simulink model "uacs_flight_bench_en"  (R2024a)
settings: Solver=ode4  StartTime=0.0  StopTime=sim_bench_t_end  FixedStep=sim_ts_ctrl  RelTol=1e-3
PreLoadFcn:
  | p=fileparts(fileparts(get_param(bdroot,'FileName')));addpath(p,fullfile(p,'params'),fullfile(p,'plant'),fullfile(p,'control'),fullfile(p,'sim'),fullfile(p,'run'),fullfile(p,'verify'),'-begin');uacs_go
PostLoadFcn:
  | uacs_bench_seed_en('uacs_flight_bench_en')
InitFcn:
  | p=fileparts(fileparts(get_param(bdroot,'FileName')));addpath(p,fullfile(p,'params'),fullfile(p,'plant'),fullfile(p,'control'),fullfile(p,'sim'),fullfile(p,'run'),fullfile(p,'verify'),'-begin');uacs_ensure
StopFcn:
  | uacs_bench_record('uacs_flight_bench_en')
undefined symbols (not defined in the file): DiscIntNeverNeededParam, sim_alpha_stall_abs, sim_c_neg1, sim_c_zero, sim_dist_gust_amp, sim_dist_gust_dir, sim_dist_gust_freq, sim_dist_wind_ned, sim_G_surf, sim_js_pitch_sign, sim_lqr_C_lat, sim_lqr_C_long, sim_lqr_K_lat, sim_lqr_K_long, sim_lqr_Tref_lat, sim_lqr_Tref_long, sim_lqr_Uff_lat, sim_lqr_Uff_long, sim_lqr_xop_lat, sim_lqr_xop_long, sim_lqr_zlim_lat, sim_lqr_zlim_lat_neg, sim_lqr_zlim_long, sim_lqr_zlim_long_neg, sim_pid_h_Dden, sim_pid_h_Dnum_abs, sim_pid_h_Isat, sim_pid_h_Isat_neg, sim_pid_h_Kp_abs, sim_pid_h_lim, sim_pid_h_lim_neg, sim_pid_h_pol, sim_pid_h_Ts, sim_pid_p_Dden, sim_pid_p_Dnum_abs, sim_pid_p_Isat, sim_pid_p_Isat_neg, sim_pid_p_Kp_abs, sim_pid_p_pol, sim_pid_p_Ts, sim_pid_phi_Dden, sim_pid_phi_Dnum_abs, sim_pid_phi_Isat, sim_pid_phi_Isat_neg, sim_pid_phi_Kp_abs, sim_pid_phi_pol, sim_pid_phi_Ts, sim_pid_q_Dden, sim_pid_q_Dnum_abs, sim_pid_q_Isat, sim_pid_q_Isat_neg, sim_pid_q_Kp_abs, sim_pid_q_pol, sim_pid_q_Ts, sim_pid_r_Dden, sim_pid_r_Dnum_abs, sim_pid_r_Isat, sim_pid_r_Isat_neg, sim_pid_r_Kp_abs, sim_pid_r_pol ... (+22)
libraries: aerolibanimutils x1
settings Model: Creator=Ash Trailer  LastModifiedBy=Ash Trailer
settings DataIOCC: SaveFormat=StructureWithTime
settings DebuggingCC: AlgebraicLoopMsg=error

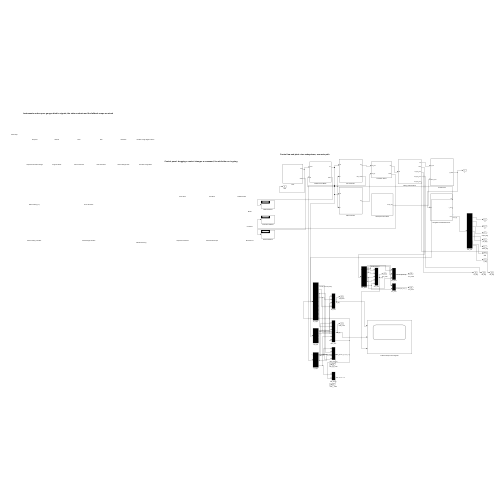
[thumbnail: Simulink's stored preview of the top-level diagram]
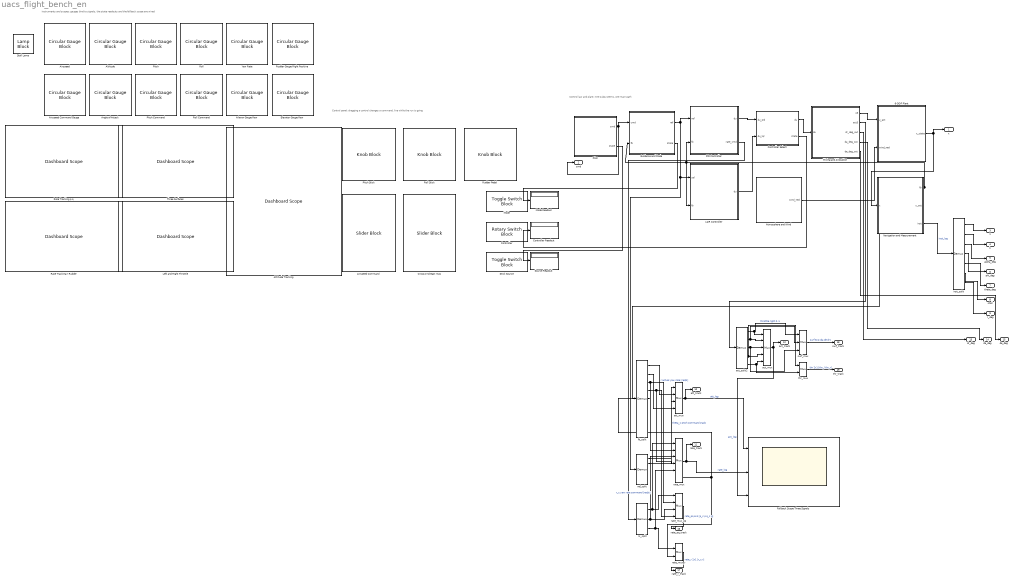
== system uacs_flight_bench_en ==
  note: Control panel: dragging a control changes a command, live while the run is going
  note: Control law and plant: nine subsystems, one main path
  note: Instruments and scopes: gauges bind to signals, the state readouts and the fallback scope are wired
  6-DOF Plant : Subsystem
  Aileron Gauge Raw : CircularGaugeBlock  ScaleMin=-30  ScaleMax=30
  Airspeed : CircularGaugeBlock  ScaleMax=40
  Airspeed Command : SliderBlock  ScaleMax=1
  Airspeed Command Gauge : CircularGaugeBlock  ScaleMax=40
  Altitude : CircularGaugeBlock  ScaleMax=400
  Angle of Attack : CircularGaugeBlock  ScaleMin=-15  ScaleMax=20
  Atmosphere and Wind : Subsystem
  Attitude Tracking : DashboardScope
  Controller : RotarySwitchBlock
      settings: Values={{'PID', 'LQR'}, [0 1]}
  Controller Readout : Display
  Controller Select : Subsystem
  Crosswind East mps : SliderBlock  ScaleMin=-10  ScaleMax=10
  Elevator Gauge Raw : CircularGaugeBlock  ScaleMin=-30  ScaleMax=30
  Fallback Scope Three Signals : Scope  NumInputPorts=3
  Guidance and Mode : Subsystem
  LQR Controller : Subsystem
  Left and Right Throttle : DashboardScope
  Mixing and Allocation : Subsystem
  Mode : ToggleSwitchBlock
      settings: Values={{'Attitude', 'Altitude'}, [0 1]}
  Mode Readout : Display
  Navigation and Measurement : Subsystem
  PID Controller : Subsystem
  Pilot : Subsystem
  Pitch : CircularGaugeBlock  ScaleMin=-30  ScaleMax=30
  Pitch Command : CircularGaugeBlock  ScaleMin=-30  ScaleMax=30
  Pitch Stick : KnobBlock  ScaleMin=-1  ScaleMax=1
  Rate Tracking p q : DashboardScope
  Rate Tracking r Rudder : DashboardScope
  Roll : CircularGaugeBlock  ScaleMin=-60  ScaleMax=60
  Roll Command : CircularGaugeBlock  ScaleMin=-60  ScaleMax=60
  Roll Stick : KnobBlock  ScaleMin=-1  ScaleMax=1
  Rudder Gauge Right Positive : CircularGaugeBlock  ScaleMin=-30  ScaleMax=30
  Rudder Pedal : KnobBlock  ScaleMin=-1  ScaleMax=1
  Source Readout : Display
  Stall Lamp : LampBlock
  Stick Source : ToggleSwitchBlock
      settings: Values={{'Virtual stick', 'Gamepad'}, [0 1]}
  Three Surfaces : DashboardScope
  Yaw Rate : CircularGaugeBlock  ScaleMin=-60  ScaleMax=60
  act_mux : Mux  Inputs=5
  act_split2 : Demux  Outputs=5
  att_mux : Mux
  fb_split : Demux  Outputs=9
  inst_split : Demux  Outputs=7
  rate_mux : Mux  Inputs=6
  rate_mux_pq : Mux
  rate_mux_r : Mux  Inputs=2
  rc_split : Demux  Outputs=3
  ref_split : Demux  Outputs=5
  surf_mux : Mux  Inputs=3
  thr_mux : Mux  Inputs=2
  x : Outport
  cmd : Outport  Port=2
  V : Outport  Port=3
  h : Outport  Port=4
  alpha_deg : Outport  Port=5
  phi_deg : Outport  Port=6
  theta_deg : Outport  Port=7
  stall : Outport  Port=8
  r_deg : Outport  Port=9
  att_track : Outport  Port=10
  rate_track : Outport  Port=11
  act_track : Outport  Port=12
  dr_deg : Outport  Port=13
  da_deg : Outport  Port=14
  de_deg : Outport  Port=15
  rate_pq_track : Outport  Port=16
  rate_r_track : Outport  Port=17
  surf_track : Outport  Port=18
  thr_track : Outport  Port=19
  wires:
  Pilot/1(cmd) -> Guidance and Mode/1(cmd), cmd/1
  Navigation and Measurement/1(fb) -> Guidance and Mode/2(fb), PID Controller/2(fb), LQR Controller/2(fb), fb_split/1
  Guidance and Mode/1(ref) -> ref_split/1, LQR Controller/1(ref), PID Controller/1(ref)
  PID Controller/1(du) -> Controller Select/1(du_pid)
  LQR Controller/1(du) -> Controller Select/2(du_lqr)
  Controller Select/1(du) -> Mixing and Allocation/1(du)
  Mixing and Allocation/1(u6) -> 6-DOF Plant/1(u_act)
  Atmosphere and Wind/1(wind_ned) -> 6-DOF Plant/2(wind_ned)
  6-DOF Plant/1(x_state) -> Navigation and Measurement/1(x), x/1
  Guidance and Mode/2(state) -> Mode Readout/1
  Controller Select/2(state) -> Controller Readout/1
  Pilot/2(state) -> Source Readout/1
  PID Controller/2(rate_cmd) -> rc_split/1
  Navigation and Measurement/3(inst) -> inst_split/1  "inst_log"
  inst_split/1 -> V/1
  inst_split/2 -> h/1
  inst_split/3 -> alpha_deg/1
  inst_split/4 -> phi_deg/1
  inst_split/5 -> theta_deg/1
  inst_split/6 -> stall/1
  inst_split/7 -> r_deg/1
  ref_split/1 -> att_mux/1  "theta_c pitch command [rad]"
  fb_split/1 -> att_mux/2  "r actual yaw rate [rad/s]"
  ref_split/2 -> att_mux/3
  fb_split/2 -> att_mux/4
  att_mux/1 -> Fallback Scope Three Signals/1, att_track/1  "att_log"
  rc_split/1 -> rate_mux/1, rate_mux_pq/1  "r_c yaw rate command [rad/s]"
  fb_split/3 -> rate_mux_pq/2, rate_mux/2
  rc_split/2 -> rate_mux/3, rate_mux_pq/3
  fb_split/4 -> rate_mux_pq/4, rate_mux/4
  rc_split/3 -> rate_mux/5, rate_mux_r/1
  fb_split/5 -> rate_mux_r/2, rate_mux/6
  rate_mux/1 -> Fallback Scope Three Signals/2, rate_track/1  "rate_log"
  Mixing and Allocation/2(act5) -> act_split2/1
  act_split2/1 -> surf_mux/1, act_mux/1  "throttle right 0..1"
  act_split2/2 -> surf_mux/2, act_mux/2
  act_split2/3 -> act_mux/3, surf_mux/3
  act_split2/4 -> act_mux/4, thr_mux/1
  act_split2/5 -> act_mux/5, thr_mux/2
  act_mux/1 -> Fallback Scope Three Signals/3, act_track/1  "act_log"
  Mixing and Allocation/3(dr_deg_out) -> dr_deg/1
  Mixing and Allocation/4(da_deg_out) -> da_deg/1
  Mixing and Allocation/5(de_deg_out) -> de_deg/1
  rate_mux_pq/1 -> rate_pq_track/1  "rate_pq 4x1 [p_c p q_c q]"
  rate_mux_r/1 -> rate_r_track/1  "rate_r 2x1 [r_c r]"
  surf_mux/1 -> surf_track/1  "surf 3x1 [da de dr]"
  thr_mux/1 -> thr_track/1  "thr 2x1 [thr_l thr_r]"

== system uacs_flight_bench_en/6-DOF Plant ==
  u_act : Inport
  wind_ned : Inport  Port=2
  plant_eom : M-S-Function  FunctionName=sim_plant_sfun
  x_state : Outport
  wires:
  u_act/1 -> plant_eom/1
  wind_ned/1 -> plant_eom/2
  plant_eom/1 -> x_state/1

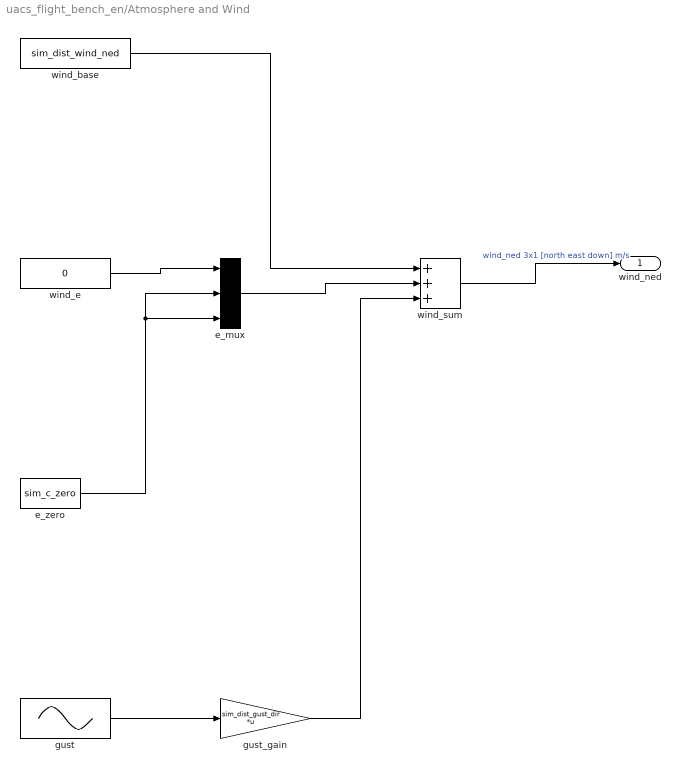
== system uacs_flight_bench_en/Atmosphere and Wind ==
  e_mux : Mux  Inputs=3
  e_zero : Constant  Value=sim_c_zero
  gust : Sin  Amplitude=sim_dist_gust_amp  Frequency=sim_dist_gust_freq  SampleTime=0
  gust_gain : Gain  Gain=sim_dist_gust_dir  Multiplication=Matrix(K*u)
  wind_base : Constant  Value=sim_dist_wind_ned
  wind_e : Constant  Value=0
  wind_sum : Sum  Inputs=+++
  wind_ned : Outport
  wires:
  wind_e/1 -> e_mux/1
  e_zero/1 -> e_mux/2, e_mux/3
  wind_base/1 -> wind_sum/1
  e_mux/1 -> wind_sum/2
  gust/1 -> gust_gain/1
  gust_gain/1 -> wind_sum/3
  wind_sum/1 -> wind_ned/1  "wind_ned 3x1 [north east down] m/s"

== system uacs_flight_bench_en/Controller Select ==
  du_pid : Inport
  du_lqr : Inport  Port=2
  k_sel : Constant  Value=0
  sw : Switch  Criteria=u2 ~= 0  Threshold=sim_c_zero  SaturateOnIntegerOverflow=off  InputSameDT=off
  du : Outport
  state : Outport  Port=2
  wires:
  du_lqr/1 -> sw/1  "1 LQR"
  k_sel/1 -> sw/2, state/1
  du_pid/1 -> sw/3  "0 PID"
  sw/1 -> du/1

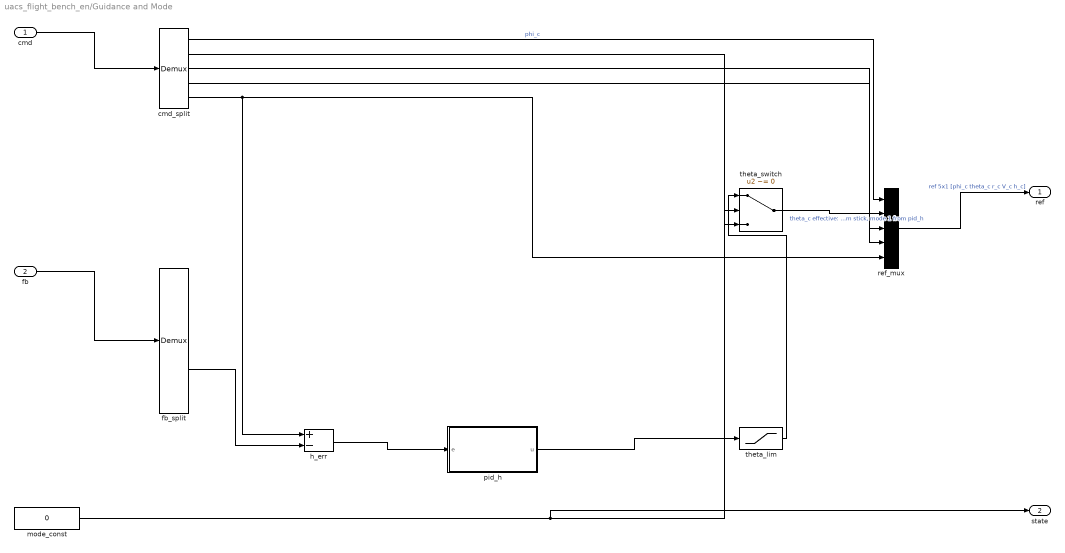
== system uacs_flight_bench_en/Guidance and Mode ==
  cmd : Inport
  fb : Inport  Port=2
  cmd_split : Demux  Outputs=5
  fb_split : Demux  Outputs=9
  h_err : Sum  Inputs=+-
  mode_const : Constant  Value=0
  pid_h : Subsystem
  ref_mux : Mux  Inputs=5
  theta_lim : Saturate  UpperLimit=sim_pid_h_lim  LowerLimit=sim_pid_h_lim_neg
  theta_switch : Switch  Criteria=u2 ~= 0  Threshold=sim_c_zero  SaturateOnIntegerOverflow=off  InputSameDT=off
  ref : Outport
  state : Outport  Port=2
  wires:
  cmd/1 -> cmd_split/1
  fb/1 -> fb_split/1
  cmd_split/5 -> h_err/1, ref_mux/5
  fb_split/7 -> h_err/2
  h_err/1 -> pid_h/1(e)
  pid_h/1(u) -> theta_lim/1
  theta_lim/1 -> theta_switch/1
  mode_const/1 -> theta_switch/2, state/1
  cmd_split/2 -> theta_switch/3
  cmd_split/1 -> ref_mux/1  "phi_c"
  theta_switch/1 -> ref_mux/2  "theta_c effective: mode 0 from stick, mode 1 from pid_h"
  cmd_split/3 -> ref_mux/3
  cmd_split/4 -> ref_mux/4
  ref_mux/1 -> ref/1  "ref 5x1 [phi_c theta_c r_c V_c h_c]"

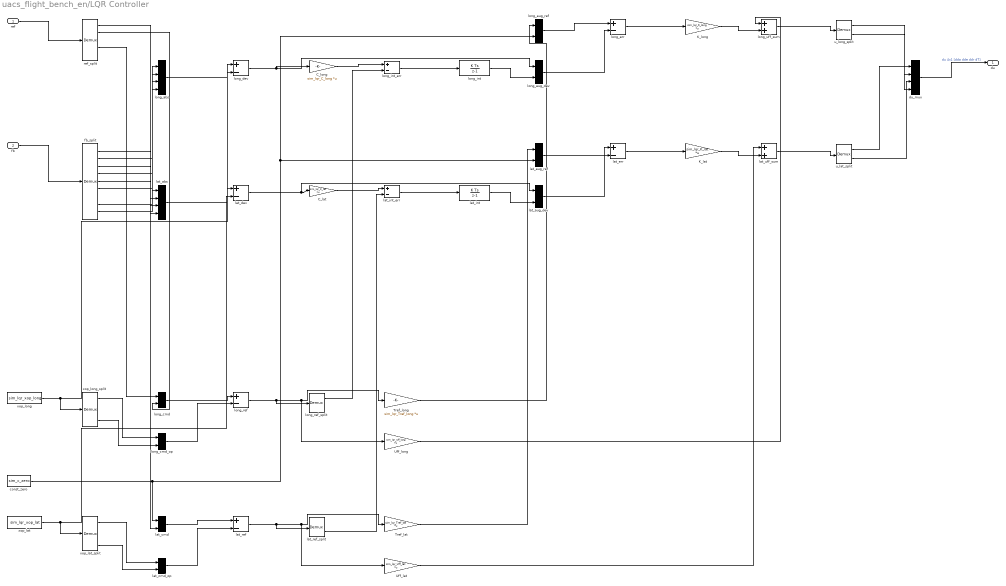
== system uacs_flight_bench_en/LQR Controller ==
  ref : Inport
  fb : Inport  Port=2
  C_lat : Gain  Gain=sim_lqr_C_lat  Multiplication=Matrix(K*u)
  C_long : Gain  Gain=sim_lqr_C_long  Multiplication=Matrix(K*u)
  K_lat : Gain  Gain=sim_lqr_K_lat  Multiplication=Matrix(K*u)
  K_long : Gain  Gain=sim_lqr_K_long  Multiplication=Matrix(K*u)
  Tref_lat : Gain  Gain=sim_lqr_Tref_lat  Multiplication=Matrix(K*u)
  Tref_long : Gain  Gain=sim_lqr_Tref_long  Multiplication=Matrix(K*u)
  Uff_lat : Gain  Gain=sim_lqr_Uff_lat  Multiplication=Matrix(K*u)
  Uff_long : Gain  Gain=sim_lqr_Uff_long  Multiplication=Matrix(K*u)
  const_zero : Constant  Value=sim_c_zero
  du_mux : Mux
  fb_split : Demux  Outputs=9
  lat_abs : Mux
  lat_aug_dev : Mux  Inputs=2
  lat_aug_ref : Mux  Inputs=2
  lat_cmd : Mux  Inputs=2
  lat_cmd_op : Mux  Inputs=2
  lat_dev : Sum  Inputs=+-
  lat_err : Sum  Inputs=+-
  lat_int : DiscreteIntegrator  gainval=sim_c_one  SampleTime=sim_ts_ctrl  LimitOutput=on  UpperSaturationLimit=sim_lqr_zlim_lat  LowerSaturationLimit=sim_lqr_zlim_lat_neg  ICPrevOutput=DiscIntNeverNeededParam  ICPrevScaledInput=DiscIntNeverNeededParam
  lat_int_err : Sum  Inputs=+-
  lat_ref : Sum  Inputs=+-
  lat_ref_split : Demux  Outputs=2
  lat_uff_sum : Sum
  long_abs : Mux
  long_aug_dev : Mux  Inputs=2
  long_aug_ref : Mux  Inputs=2
  long_cmd : Mux  Inputs=2
  long_cmd_op : Mux  Inputs=2
  long_dev : Sum  Inputs=+-
  long_err : Sum  Inputs=+-
  long_int : DiscreteIntegrator  gainval=sim_c_one  SampleTime=sim_ts_ctrl  LimitOutput=on  UpperSaturationLimit=sim_lqr_zlim_long  LowerSaturationLimit=sim_lqr_zlim_long_neg  ICPrevOutput=DiscIntNeverNeededParam  ICPrevScaledInput=DiscIntNeverNeededParam
  long_int_err : Sum  Inputs=+-
  long_ref : Sum  Inputs=+-
  long_ref_split : Demux  Outputs=2
  long_uff_sum : Sum
  ref_split : Demux  Outputs=5
  u_lat_split : Demux  Outputs=2
  u_long_split : Demux  Outputs=2
  xop_lat : Constant  Value=sim_lqr_xop_lat
  xop_lat_split : Demux
  xop_long : Constant  Value=sim_lqr_xop_long
  xop_long_split : Demux
  du : Outport
  wires:
  ref/1 -> ref_split/1
  fb/1 -> fb_split/1
  xop_long/1 -> xop_long_split/1, long_dev/2
  xop_lat/1 -> xop_lat_split/1, lat_dev/2
  ref_split/4 -> long_cmd/1
  ref_split/2 -> long_cmd/2
  xop_long_split/1 -> long_cmd_op/1
  xop_long_split/4 -> long_cmd_op/2
  long_cmd/1 -> long_ref/1
  long_cmd_op/1 -> long_ref/2
  long_ref/1 -> Tref_long/1, Uff_long/1, long_ref_split/1
  const_zero/1 -> long_aug_ref/2, lat_aug_ref/2, lat_cmd/1
  ref_split/1 -> lat_cmd/2
  xop_lat_split/1 -> lat_cmd_op/1
  xop_lat_split/4 -> lat_cmd_op/2
  lat_cmd/1 -> lat_ref/1
  lat_cmd_op/1 -> lat_ref/2
  lat_ref/1 -> Tref_lat/1, Uff_lat/1, lat_ref_split/1
  fb_split/6 -> long_abs/1
  fb_split/8 -> long_abs/2
  fb_split/4 -> long_abs/3
  fb_split/2 -> long_abs/4
  long_abs/1 -> long_dev/1
  long_dev/1 -> C_long/1, long_aug_dev/1
  C_long/1 -> long_int_err/1
  long_ref_split/1 -> long_int_err/2
  long_int_err/1 -> long_int/1
  long_int/1 -> long_aug_dev/2
  Tref_long/1 -> long_aug_ref/1
  long_aug_ref/1 -> long_err/1
  long_aug_dev/1 -> long_err/2
  long_err/1 -> K_long/1
  K_long/1 -> long_uff_sum/2
  Uff_long/1 -> long_uff_sum/1
  long_uff_sum/1 -> u_long_split/1
  fb_split/9 -> lat_abs/1
  fb_split/3 -> lat_abs/2
  fb_split/5 -> lat_abs/3
  fb_split/1 -> lat_abs/4
  lat_abs/1 -> lat_dev/1
  lat_dev/1 -> C_lat/1, lat_aug_dev/1
  C_lat/1 -> lat_int_err/1
  lat_ref_split/2 -> lat_int_err/2
  lat_int_err/1 -> lat_int/1
  lat_int/1 -> lat_aug_dev/2
  Tref_lat/1 -> lat_aug_ref/1
  lat_aug_ref/1 -> lat_err/1
  lat_aug_dev/1 -> lat_err/2
  lat_err/1 -> K_lat/1
  K_lat/1 -> lat_uff_sum/2
  Uff_lat/1 -> lat_uff_sum/1
  lat_uff_sum/1 -> u_lat_split/1
  u_lat_split/1 -> du_mux/1
  u_long_split/1 -> du_mux/2
  u_lat_split/2 -> du_mux/3
  u_long_split/2 -> du_mux/4
  du_mux/1 -> du/1  "du 4x1 [dda dde ddr dT]"

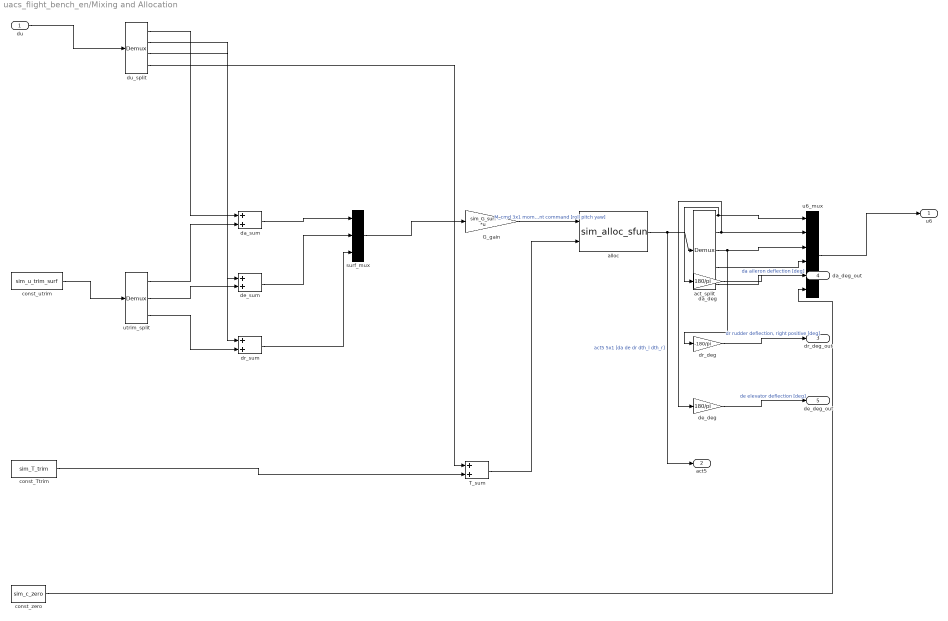
== system uacs_flight_bench_en/Mixing and Allocation ==
  du : Inport
  G_gain : Gain  Gain=sim_G_surf  Multiplication=Matrix(K*u)
  T_sum : Sum
  act_split : Demux  Outputs=5
  alloc : M-S-Function  FunctionName=sim_alloc_sfun
  const_Ttrim : Constant  Value=sim_T_trim
  const_utrim : Constant  Value=sim_u_trim_surf
  const_zero : Constant  Value=sim_c_zero
  da_deg : Gain  Gain=180/pi
  da_sum : Sum
  de_deg : Gain  Gain=180/pi
  de_sum : Sum
  dr_deg : Gain  Gain=-180/pi
  dr_sum : Sum
  du_split : Demux
  surf_mux : Mux  Inputs=3
  u6_mux : Mux  Inputs=6
  utrim_split : Demux  Outputs=3
  u6 : Outport
  act5 : Outport  Port=2
  dr_deg_out : Outport  Port=3
  da_deg_out : Outport  Port=4
  de_deg_out : Outport  Port=5
  wires:
  act_split/1 -> da_deg/1, u6_mux/1
  da_deg/1 -> da_deg_out/1  "da aileron deflection [deg]"
  act_split/2 -> de_deg/1, u6_mux/2
  de_deg/1 -> de_deg_out/1  "de elevator deflection [deg]"
  act_split/3 -> dr_deg/1, u6_mux/3
  dr_deg/1 -> dr_deg_out/1  "dr rudder deflection, right positive [deg]"
  du/1 -> du_split/1
  const_utrim/1 -> utrim_split/1
  du_split/1 -> da_sum/1
  utrim_split/1 -> da_sum/2
  du_split/2 -> de_sum/1
  utrim_split/2 -> de_sum/2
  du_split/3 -> dr_sum/1
  utrim_split/3 -> dr_sum/2
  da_sum/1 -> surf_mux/1
  de_sum/1 -> surf_mux/2
  dr_sum/1 -> surf_mux/3
  surf_mux/1 -> G_gain/1
  G_gain/1 -> alloc/1  "M_cmd 3x1 moment command [roll pitch yaw]"
  du_split/4 -> T_sum/1
  const_Ttrim/1 -> T_sum/2
  T_sum/1 -> alloc/2
  alloc/1 -> act_split/1, act5/1  "act5 5x1 [da de dr dth_l dth_r]"
  act_split/4 -> u6_mux/4
  act_split/5 -> u6_mux/5
  const_zero/1 -> u6_mux/6
  u6_mux/1 -> u6/1

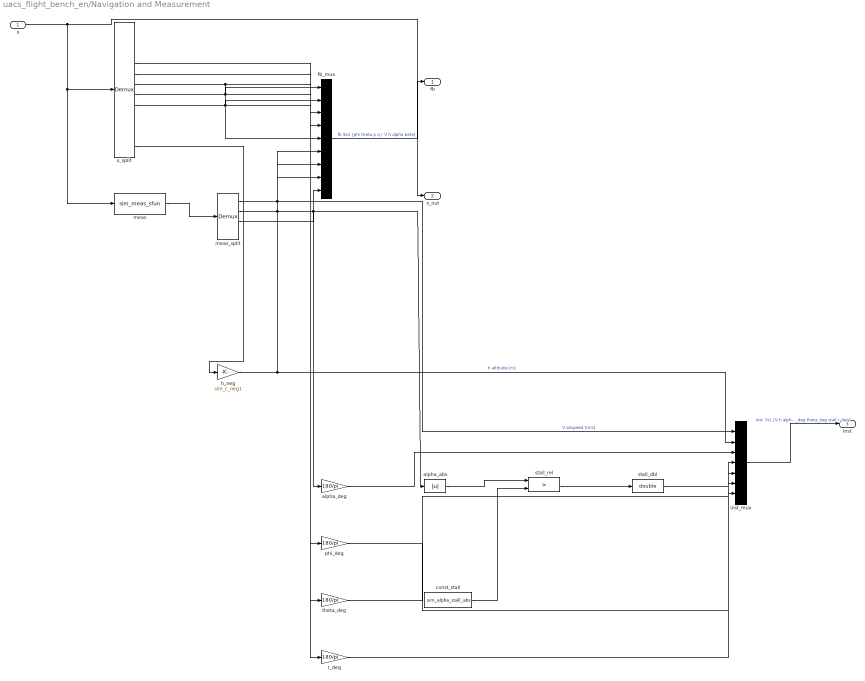
== system uacs_flight_bench_en/Navigation and Measurement ==
  x : Inport
  alpha_abs : Abs  SaturateOnIntegerOverflow=off
  alpha_deg : Gain  Gain=180/pi
  const_stall : Constant  Value=sim_alpha_stall_abs
  fb_mux : Mux  Inputs=9
  h_neg : Gain  Gain=sim_c_neg1
  inst_mux : Mux  Inputs=7
  meas : M-S-Function  FunctionName=sim_meas_sfun
  meas_split : Demux
  phi_deg : Gain  Gain=180/pi
  r_deg : Gain  Gain=180/pi
  stall_dbl : DataTypeConversion  OutDataTypeStr=double  SaturateOnIntegerOverflow=off  RndMeth=Floor
  stall_rel : RelationalOperator  Operator=>  OutDataTypeStr=boolean  RndMeth=Simplest  InputSameDT=off
  theta_deg : Gain  Gain=180/pi
  x_split : Demux  Outputs=12
  fb : Outport
  x_out : Outport  Port=2
  inst : Outport  Port=3
  wires:
  x/1 -> x_split/1, meas/1, x_out/1
  meas/1 -> meas_split/1
  x_split/12 -> h_neg/1
  meas_split/2 -> alpha_deg/1, alpha_abs/1, fb_mux/8
  alpha_abs/1 -> stall_rel/1
  const_stall/1 -> stall_rel/2
  stall_rel/1 -> stall_dbl/1
  x_split/7 -> phi_deg/1, fb_mux/1
  x_split/8 -> theta_deg/1, fb_mux/2
  x_split/6 -> r_deg/1, fb_mux/5
  meas_split/1 -> inst_mux/1, fb_mux/6  "V airspeed [m/s]"
  h_neg/1 -> inst_mux/2, fb_mux/7  "h altitude [m]"
  alpha_deg/1 -> inst_mux/3
  phi_deg/1 -> inst_mux/4
  theta_deg/1 -> inst_mux/5
  stall_dbl/1 -> inst_mux/6
  r_deg/1 -> inst_mux/7
  inst_mux/1 -> inst/1  "inst 7x1 [V h alpha_deg phi_deg theta_deg stall r_deg]"
  x_split/4 -> fb_mux/3
  x_split/5 -> fb_mux/4
  meas_split/3 -> fb_mux/9
  fb_mux/1 -> fb/1  "fb 9x1 [phi theta p q r V h alpha beta]"

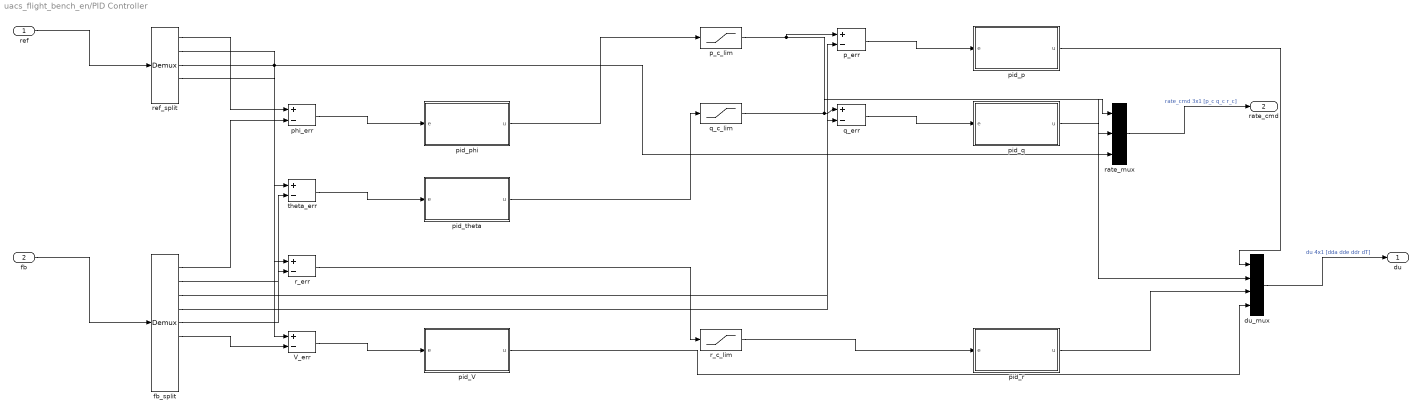
== system uacs_flight_bench_en/PID Controller ==
  ref : Inport
  fb : Inport  Port=2
  V_err : Sum  Inputs=+-
  du_mux : Mux
  fb_split : Demux  Outputs=9
  p_c_lim : Saturate  UpperLimit=sim_rate_cmd_lim_p  LowerLimit=-sim_rate_cmd_lim_p
  p_err : Sum  Inputs=+-
  phi_err : Sum  Inputs=+-
  pid_V : Subsystem
  pid_p : Subsystem
  pid_phi : Subsystem
  pid_q : Subsystem
  pid_r : Subsystem
  pid_theta : Subsystem
  q_c_lim : Saturate  UpperLimit=sim_rate_cmd_lim_q  LowerLimit=-sim_rate_cmd_lim_q
  q_err : Sum  Inputs=+-
  r_c_lim : Saturate  UpperLimit=sim_rate_cmd_lim_r  LowerLimit=-sim_rate_cmd_lim_r
  r_err : Sum  Inputs=+-
  rate_mux : Mux  Inputs=3
  ref_split : Demux  Outputs=5
  theta_err : Sum  Inputs=+-
  du : Outport
  rate_cmd : Outport  Port=2
  wires:
  ref/1 -> ref_split/1
  fb/1 -> fb_split/1
  ref_split/1 -> phi_err/1
  fb_split/1 -> phi_err/2
  phi_err/1 -> pid_phi/1(e)
  pid_phi/1(u) -> p_c_lim/1
  ref_split/2 -> theta_err/1
  fb_split/2 -> theta_err/2
  theta_err/1 -> pid_theta/1(e)
  pid_theta/1(u) -> q_c_lim/1
  ref_split/3 -> r_err/1, rate_mux/3
  fb_split/5 -> r_err/2
  r_err/1 -> r_c_lim/1
  r_c_lim/1 -> pid_r/1(e)
  ref_split/4 -> V_err/1
  fb_split/6 -> V_err/2
  V_err/1 -> pid_V/1(e)
  p_c_lim/1 -> p_err/1, rate_mux/1
  fb_split/3 -> p_err/2
  p_err/1 -> pid_p/1(e)
  q_c_lim/1 -> q_err/1, rate_mux/2
  fb_split/4 -> q_err/2
  q_err/1 -> pid_q/1(e)
  rate_mux/1 -> rate_cmd/1  "rate_cmd 3x1 [p_c q_c r_c]"
  pid_p/1(u) -> du_mux/1
  pid_q/1(u) -> du_mux/2
  pid_r/1(u) -> du_mux/3
  pid_V/1(u) -> du_mux/4
  du_mux/1 -> du/1  "du 4x1 [dda dde ddr dT]"

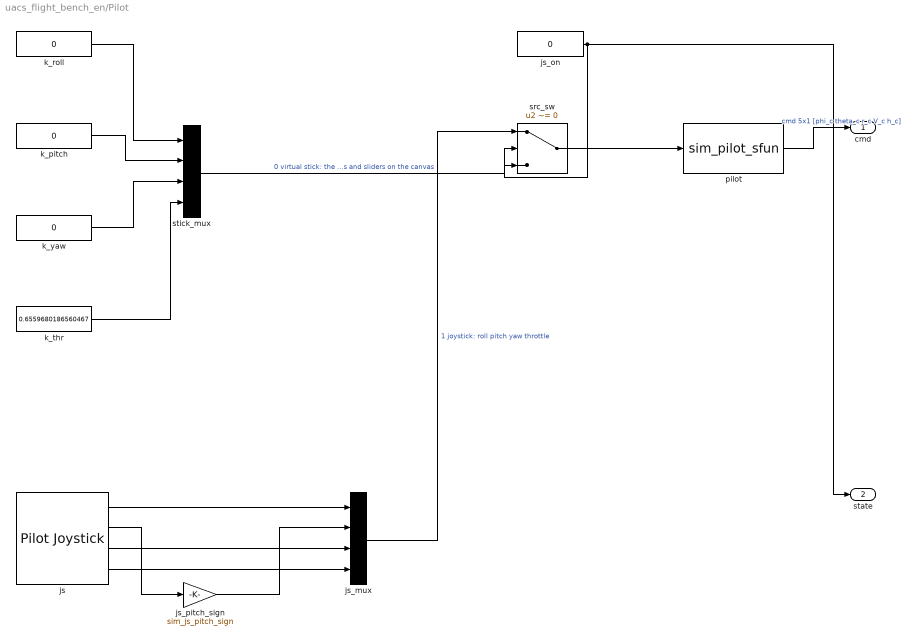
== system uacs_flight_bench_en/Pilot ==
  js : aerolibanimutils/Pilot Joystick  JoystickID=None  OutputConfiguration=FourAxis  SampleTime=sim_ts_outer
  js_mux : Mux
  js_on : Constant  Value=0
  js_pitch_sign : Gain  Gain=sim_js_pitch_sign
  k_pitch : Constant  Value=0
  k_roll : Constant  Value=0
  k_thr : Constant  Value=0.6559680186560467
  k_yaw : Constant  Value=0
  pilot : M-S-Function  FunctionName=sim_pilot_sfun
  src_sw : Switch  Criteria=u2 ~= 0  Threshold=sim_c_zero  SaturateOnIntegerOverflow=off  InputSameDT=off
  stick_mux : Mux
  cmd : Outport
  state : Outport  Port=2
  wires:
  k_roll/1 -> stick_mux/1
  k_pitch/1 -> stick_mux/2
  k_yaw/1 -> stick_mux/3
  k_thr/1 -> stick_mux/4
  js/1 -> js_mux/1
  js/2 -> js_pitch_sign/1
  js_pitch_sign/1 -> js_mux/2
  js/3 -> js_mux/3
  js/4 -> js_mux/4
  js_mux/1 -> src_sw/1  "1 joystick: roll pitch yaw throttle"
  js_on/1 -> src_sw/2, state/1
  stick_mux/1 -> src_sw/3  "0 virtual stick: the knobs and sliders on the canvas"
  src_sw/1 -> pilot/1
  pilot/1 -> cmd/1  "cmd 5x1 [phi_c theta_c r_c V_c h_c]"

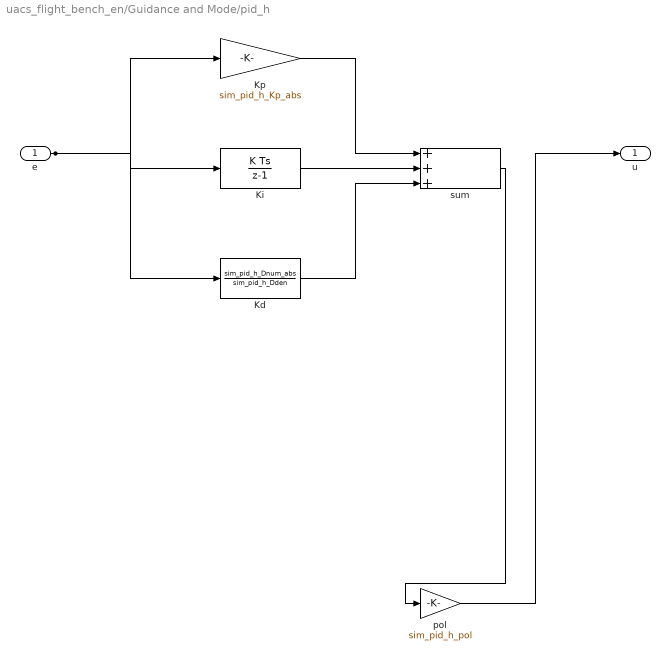
== system uacs_flight_bench_en/Guidance and Mode/pid_h ==
  e : Inport
  Kd : DiscreteTransferFcn  Numerator=sim_pid_h_Dnum_abs  Denominator=sim_pid_h_Dden  SampleTime=sim_pid_h_Ts
  Ki : DiscreteIntegrator  gainval=sim_pid_h_Ki_abs  SampleTime=sim_pid_h_Ts  LimitOutput=on  UpperSaturationLimit=sim_pid_h_Isat  LowerSaturationLimit=sim_pid_h_Isat_neg  ICPrevOutput=DiscIntNeverNeededParam  ICPrevScaledInput=DiscIntNeverNeededParam
  Kp : Gain  Gain=sim_pid_h_Kp_abs
  pol : Gain  Gain=sim_pid_h_pol
  sum : Sum  Inputs=+++
  u : Outport
  wires:
  e/1 -> Kp/1, Ki/1, Kd/1
  Kp/1 -> sum/1
  Ki/1 -> sum/2
  Kd/1 -> sum/3
  sum/1 -> pol/1
  pol/1 -> u/1

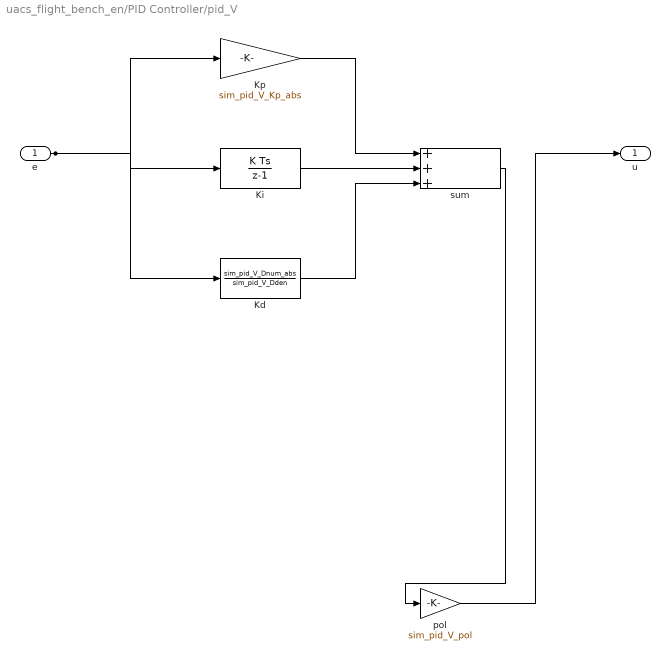
== system uacs_flight_bench_en/PID Controller/pid_V ==
  e : Inport
  Kd : DiscreteTransferFcn  Numerator=sim_pid_V_Dnum_abs  Denominator=sim_pid_V_Dden  SampleTime=sim_pid_V_Ts
  Ki : DiscreteIntegrator  gainval=sim_pid_V_Ki_abs  SampleTime=sim_pid_V_Ts  LimitOutput=on  UpperSaturationLimit=sim_pid_V_Isat  LowerSaturationLimit=sim_pid_V_Isat_neg  ICPrevOutput=DiscIntNeverNeededParam  ICPrevScaledInput=DiscIntNeverNeededParam
  Kp : Gain  Gain=sim_pid_V_Kp_abs
  pol : Gain  Gain=sim_pid_V_pol
  sum : Sum  Inputs=+++
  u : Outport
  wires:
  e/1 -> Kp/1, Ki/1, Kd/1
  Kp/1 -> sum/1
  Ki/1 -> sum/2
  Kd/1 -> sum/3
  sum/1 -> pol/1
  pol/1 -> u/1

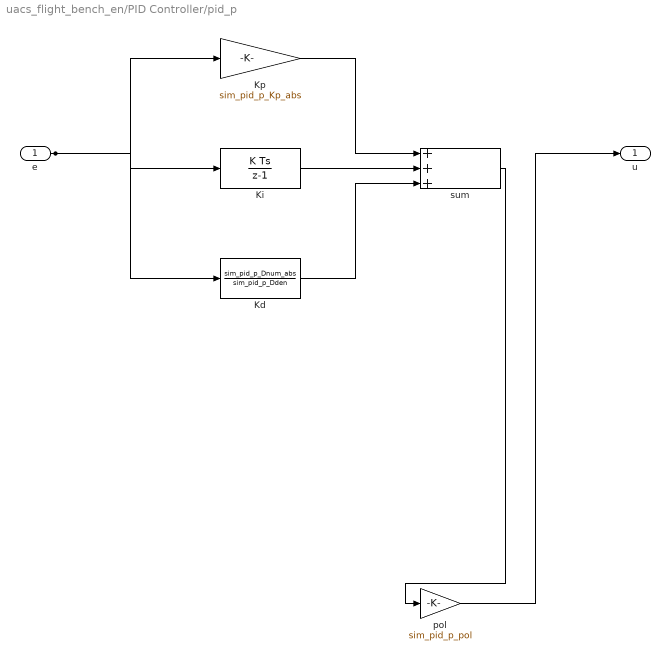
== system uacs_flight_bench_en/PID Controller/pid_p ==
  e : Inport
  Kd : DiscreteTransferFcn  Numerator=sim_pid_p_Dnum_abs  Denominator=sim_pid_p_Dden  SampleTime=sim_pid_p_Ts
  Ki : DiscreteIntegrator  gainval=sim_pid_p_Ki_abs  SampleTime=sim_pid_p_Ts  LimitOutput=on  UpperSaturationLimit=sim_pid_p_Isat  LowerSaturationLimit=sim_pid_p_Isat_neg  ICPrevOutput=DiscIntNeverNeededParam  ICPrevScaledInput=DiscIntNeverNeededParam
  Kp : Gain  Gain=sim_pid_p_Kp_abs
  pol : Gain  Gain=sim_pid_p_pol
  sum : Sum  Inputs=+++
  u : Outport
  wires:
  e/1 -> Kp/1, Ki/1, Kd/1
  Kp/1 -> sum/1
  Ki/1 -> sum/2
  Kd/1 -> sum/3
  sum/1 -> pol/1
  pol/1 -> u/1

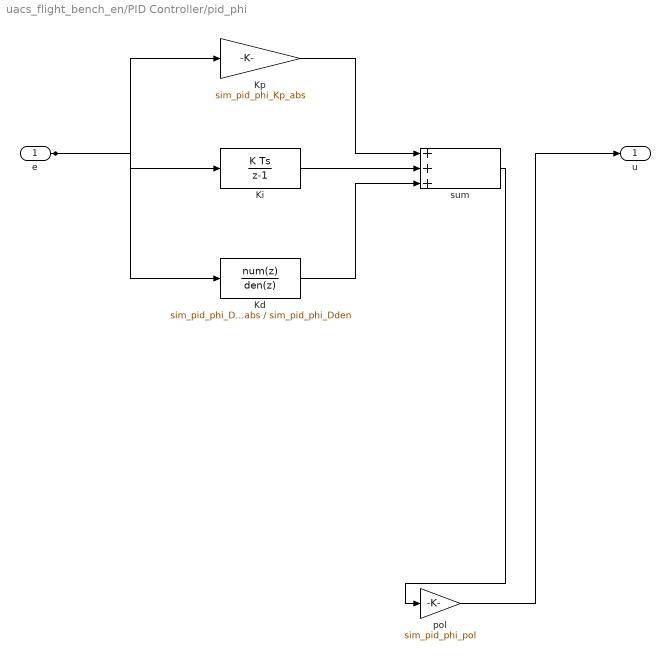
== system uacs_flight_bench_en/PID Controller/pid_phi ==
  e : Inport
  Kd : DiscreteTransferFcn  Numerator=sim_pid_phi_Dnum_abs  Denominator=sim_pid_phi_Dden  SampleTime=sim_pid_phi_Ts
  Ki : DiscreteIntegrator  gainval=sim_pid_phi_Ki_abs  SampleTime=sim_pid_phi_Ts  LimitOutput=on  UpperSaturationLimit=sim_pid_phi_Isat  LowerSaturationLimit=sim_pid_phi_Isat_neg  ICPrevOutput=DiscIntNeverNeededParam  ICPrevScaledInput=DiscIntNeverNeededParam
  Kp : Gain  Gain=sim_pid_phi_Kp_abs
  pol : Gain  Gain=sim_pid_phi_pol
  sum : Sum  Inputs=+++
  u : Outport
  wires:
  e/1 -> Kp/1, Ki/1, Kd/1
  Kp/1 -> sum/1
  Ki/1 -> sum/2
  Kd/1 -> sum/3
  sum/1 -> pol/1
  pol/1 -> u/1

== system uacs_flight_bench_en/PID Controller/pid_q ==
  e : Inport
  Kd : DiscreteTransferFcn  Numerator=sim_pid_q_Dnum_abs  Denominator=sim_pid_q_Dden  SampleTime=sim_pid_q_Ts
  Ki : DiscreteIntegrator  gainval=sim_pid_q_Ki_abs  SampleTime=sim_pid_q_Ts  LimitOutput=on  UpperSaturationLimit=sim_pid_q_Isat  LowerSaturationLimit=sim_pid_q_Isat_neg  ICPrevOutput=DiscIntNeverNeededParam  ICPrevScaledInput=DiscIntNeverNeededParam
  Kp : Gain  Gain=sim_pid_q_Kp_abs
  pol : Gain  Gain=sim_pid_q_pol
  sum : Sum  Inputs=+++
  u : Outport
  wires:
  e/1 -> Kp/1, Ki/1, Kd/1
  Kp/1 -> sum/1
  Ki/1 -> sum/2
  Kd/1 -> sum/3
  sum/1 -> pol/1
  pol/1 -> u/1

== system uacs_flight_bench_en/PID Controller/pid_r ==
  e : Inport
  Kd : DiscreteTransferFcn  Numerator=sim_pid_r_Dnum_abs  Denominator=sim_pid_r_Dden  SampleTime=sim_pid_r_Ts
  Ki : DiscreteIntegrator  gainval=sim_pid_r_Ki_abs  SampleTime=sim_pid_r_Ts  LimitOutput=on  UpperSaturationLimit=sim_pid_r_Isat  LowerSaturationLimit=sim_pid_r_Isat_neg  ICPrevOutput=DiscIntNeverNeededParam  ICPrevScaledInput=DiscIntNeverNeededParam
  Kp : Gain  Gain=sim_pid_r_Kp_abs
  pol : Gain  Gain=sim_pid_r_pol
  sum : Sum  Inputs=+++
  u : Outport
  wires:
  e/1 -> Kp/1, Ki/1, Kd/1
  Kp/1 -> sum/1
  Ki/1 -> sum/2
  Kd/1 -> sum/3
  sum/1 -> pol/1
  pol/1 -> u/1

== system uacs_flight_bench_en/PID Controller/pid_theta ==
  e : Inport
  Kd : DiscreteTransferFcn  Numerator=sim_pid_theta_Dnum_abs  Denominator=sim_pid_theta_Dden  SampleTime=sim_pid_theta_Ts
  Ki : DiscreteIntegrator  gainval=sim_pid_theta_Ki_abs  SampleTime=sim_pid_theta_Ts  LimitOutput=on  UpperSaturationLimit=sim_pid_theta_Isat  LowerSaturationLimit=sim_pid_theta_Isat_neg  ICPrevOutput=DiscIntNeverNeededParam  ICPrevScaledInput=DiscIntNeverNeededParam
  Kp : Gain  Gain=sim_pid_theta_Kp_abs
  pol : Gain  Gain=sim_pid_theta_pol
  sum : Sum  Inputs=+++
  u : Outport
  wires:
  e/1 -> Kp/1, Ki/1, Kd/1
  Kp/1 -> sum/1
  Ki/1 -> sum/2
  Kd/1 -> sum/3
  sum/1 -> pol/1
  pol/1 -> u/1
